simulink model "Pendulum_Simulink"  (R2025b)
settings: Solver=VariableStepAuto  StopTime=30
InitFcn:
  | InvertedPendulum
values from neighbouring files (symbols this model uses):
  G0_den = [1 b -K]    [InvertedPendulum.m]
  G0_num = [0 0 c]    [InvertedPendulum.m]
undefined symbols (not defined in the file or in its folder): C_den, C_num, dist_angle
libraries: simulink x2
settings Model: Creator=slaga  LastModifiedBy=slaga
settings SFSimCC: SimGPUStackLimitPerThread=51200  SimGPUMallocThreshold=200
settings RTWCC: GPUStackLimitPerThread=51200  GPUMallocThreshold=200

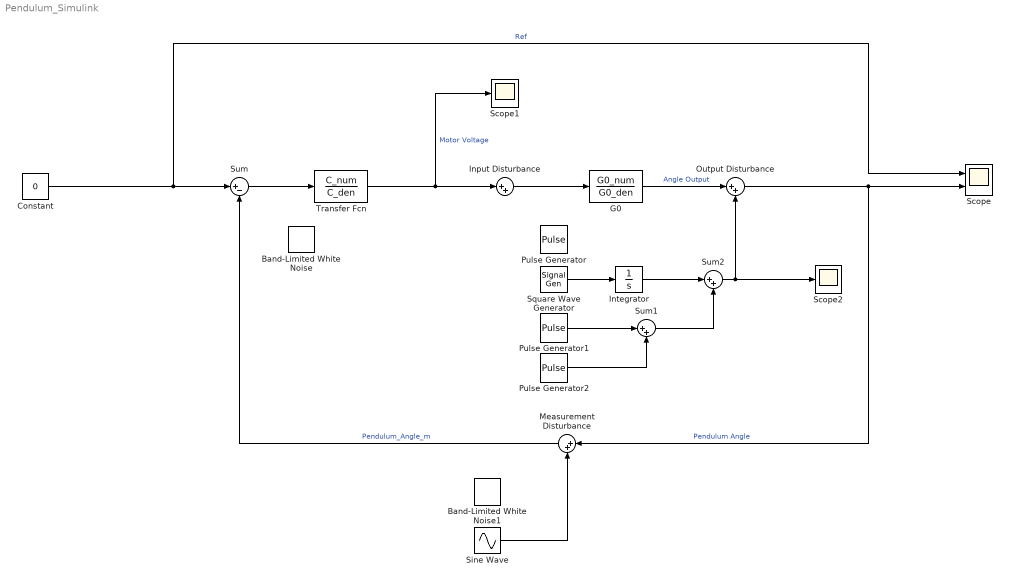
== system Pendulum_Simulink ==
  Band-Limited White Noise : simulink/Sources/Band-Limited White Noise  Cov=[0.01]  Ts=0.1  seed=[23341]
  Band-Limited White Noise1 : simulink/Sources/Band-Limited White Noise  Cov=[0.01]  Ts=0.1  seed=[23341]
  Constant : Constant  Value=0
  G0 : TransferFcn  Numerator=G0_num  Denominator=G0_den
  Input Disturbance : Sum  Inputs=|++
  Integrator : Integrator
  Measurement Disturbance : Sum  Inputs=|++
  Output Disturbance : Sum  Inputs=|++
  Pulse Generator : DiscretePulseGenerator  PulseType=Time based  Amplitude=(pi/180)*dist_angle  Period=100  PulseWidth=0.01  PhaseDelay=1
  Pulse Generator1 : DiscretePulseGenerator  PulseType=Time based  Amplitude=10  Period=6  PulseWidth=0.1  PhaseDelay=3
  Pulse Generator2 : DiscretePulseGenerator  PulseType=Time based  Amplitude=-10  Period=6  PulseWidth=0.1
  Scope : Scope  NumInputPorts=2
      settings: ActiveDisplayYMinimum=-11.487529265527863  ActiveDisplayYMaximum=10.142974196506495
  Scope1 : Scope
      settings: ActiveDisplayYMinimum=-87265.145820986552  ActiveDisplayYMaximum=83221.330431747992
  Scope2 : Scope
      settings: ActiveDisplayYMinimum=-12.111549484921074  ActiveDisplayYMaximum=8.97111745661654  DataLoggingVariableName=ScopeData2
  Sine Wave : Sin  Amplitude=0.1  Frequency=100  SampleTime=0
  Square Wave Generator : SignalGenerator  WaveForm=square  Amplitude=pi/3  Frequency=1/6
  Sum : Sum  Inputs=|+-
  Sum1 : Sum  Inputs=|++
  Sum2 : Sum  Inputs=|++
  Transfer Fcn : TransferFcn  Numerator=C_num  Denominator=C_den
  wires:
  Sum/1 -> Transfer Fcn/1
  Constant/1 -> Scope/1, Sum/1  "Ref"
  G0/1 -> Output Disturbance/1  "Angle Output"
  Output Disturbance/1 -> Measurement Disturbance/1, Scope/2  "Pendulum Angle"
  Input Disturbance/1 -> G0/1
  Transfer Fcn/1 -> Scope1/1, Input Disturbance/1  "Motor Voltage"
  Measurement Disturbance/1 -> Sum/2  "Pendulum_Angle_m"
  Sine Wave/1 -> Measurement Disturbance/2
  Square Wave Generator/1 -> Integrator/1
  Pulse Generator1/1 -> Sum1/1
  Pulse Generator2/1 -> Sum1/2
  Integrator/1 -> Sum2/1
  Sum1/1 -> Sum2/2
  Sum2/1 -> Scope2/1, Output Disturbance/2
